simulink model "ErrorFeedback"  (R2025b)
settings: Solver=ode45  StartTime=0.0  StopTime=10.0  RelTol=1e-3
settings Model: Creator=Ishwar  LastModifiedBy=Ishwar

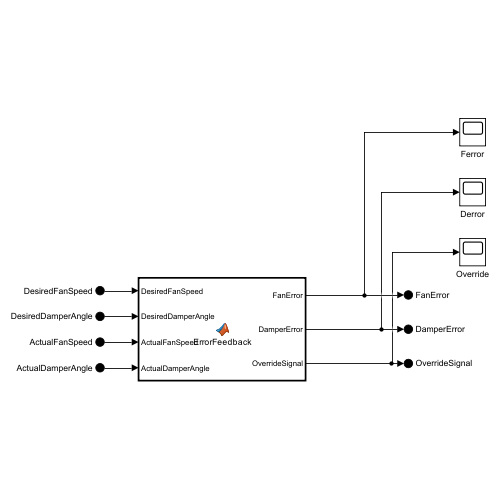
[thumbnail: Simulink's stored preview of the top-level diagram]
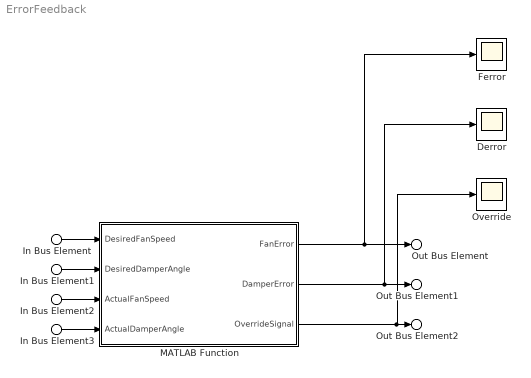
== system ErrorFeedback ==
  In Bus Element : Inport  PortName=DesiredFanSpeed
  In Bus Element1 : Inport  Port=2  PortName=DesiredDamperAngle
  In Bus Element3 : Inport  Port=3  PortName=ActualDamperAngle
  In Bus Element2 : Inport  Port=4  PortName=ActualFanSpeed
  Derror : Scope
      settings: ActiveDisplayYMinimum=-15.984583333333342  ActiveDisplayYMaximum=-3.4845833333333407
  Ferror : Scope
      settings: ActiveDisplayYMinimum=5.98458333333334  ActiveDisplayYMaximum=13.484583333333342
  MATLAB Function : MATLAB Function  TreatAsAtomicUnit=on
  Override : Scope
      settings: ActiveDisplayYMinimum=0.8831176026570049  ActiveDisplayYMaximum=1.1146426026570049  DataLoggingVariableName=ScopeData2
  Out Bus Element : Outport  PortName=FanError
  Out Bus Element1 : Outport  Port=2  PortName=DamperError
  Out Bus Element2 : Outport  Port=3  PortName=OverrideSignal
  wires:
  In Bus Element/1 -> MATLAB Function/1(DesiredFanSpeed)
  In Bus Element1/1 -> MATLAB Function/2(DesiredDamperAngle)
  In Bus Element2/1 -> MATLAB Function/3(ActualFanSpeed)
  In Bus Element3/1 -> MATLAB Function/4(ActualDamperAngle)
  MATLAB Function/2(DamperError) -> Derror/1, Out Bus Element1/1
  MATLAB Function/1(FanError) -> Ferror/1, Out Bus Element/1
  MATLAB Function/3(OverrideSignal) -> Override/1, Out Bus Element2/1

== matlab function ErrorFeedback/MATLAB Function ==
  data: DesiredFanSpeed input; FanError output; DesiredDamperAngle input; ActualFanSpeed input; ActualDamperAngle input; DamperError output; OverrideSignal output
function [FanError, DamperError, OverrideSignal] = ErrorFeedback(DesiredFanSpeed, DesiredDamperAngle, ActualFanSpeed, ActualDamperAngle)
%#codegen

% Thresholds
thresholdFan = 5;     % allowable deviation in %
thresholdDamper = 5;   % allowable deviation in degrees

% Error calculations (double by default)
FanError    = DesiredFanSpeed - ActualFanSpeed;
DamperError = DesiredDamperAngle - ActualDamperAngle;

% Override logic (keep as double to match Simulink ports)
if abs(FanError) > thresholdFan || abs(DamperError) > thresholdDamper
    OverrideSignal = 1;   % double
else
    OverrideSignal = 0;   % double
end
